simulink model "ps_model"  (R2025b)
settings: Solver=ode23tb  StartTime=0.0  StopTime=simlength  FixedStep=tc  MaxStep=tc
values from neighbouring files (symbols this model uses):
  omega_grid_emulator_nom = w_grid    (= 314.159265359)    [grid_emulator.m]
  omega_grid_nom = w_grid    (= 314.159265359)    [grid_emulator.m]
  ugrid_factor = 1    [grid_emulator.m]
  V_phase_normalization_factor = Vgrid_phase_normalization_factor    [grid_emulator.m]
  Vdc_base = 720    [grid_emulator.m]
  vn_eta_pu = 0    [grid_emulator.m]
  vn_xi_pu = 0    [grid_emulator.m]
  vp_xi_pu = 1    [grid_emulator.m]
undefined symbols (not defined in the file or in its folder): CFi, fnom, fPWM_INV, i_nom, ki_i, ki_u, kp_i, kp_u, Ld2_trafo_out, magnitude, n10, number_of_cells, omega_nom, Q, q1Kalman, q2Kalman, q3Kalman, R_RLload, Rd2_trafo_out, rKalman, tc, time_load_step, ts_afe, ts_inv, tsample, u_nom, Vdc_nom
libraries: fl_lib x120, nesl_utility x67, ee_lib x7, cstblocks x4, moving_average_filter x4, single_phase_transformer_lib x3, lithium_ion_cell_lib x1, simulink x1, threephase_inductor_lib x1
(part 4 of 4)

== system ps_model/inverter/MOS based inverter/spwm/modulator1/PWM generator 3 ==
  m_index : Inport
  phase : Inport  Port=2
  Clock : Clock
  Constant : Constant  Value=dead_time*f
  Constant1 : Constant  Value=polarity
  Constant2 : Constant  Value=1/f
  Constant4 : Constant
  Data Type Conversion1 : DataTypeConversion
  Data Type Conversion2 : DataTypeConversion
  Gain4 : Gain  Gain=1/2
  Gain5 : Gain  Gain=1/(pi/2)
  Hit Crossing : HitCross  ShowOutputPort=off
  Hit Crossing1 : HitCross  ShowOutputPort=off
  MATLAB Function : MATLAB Function  TreatAsAtomicUnit=on
  Relational Operator1 : RelationalOperator  Operator=<=  InputSameDT=off
  Relational Operator2 : RelationalOperator  Operator=<=  InputSameDT=off
  Relay : Relay  OnOutputValue=pos_cmd_gate  OffOutputValue=neg_cmd_gate
  Relay1 : Relay  OnOutputValue=pos_cmd_gate  OffOutputValue=neg_cmd_gate
  Saturation1 : Saturate  UpperLimit=m_up  LowerLimit=m_low
  Sum : Sum  Inputs=|++  SaturateOnIntegerOverflow=on
  Sum1 : Sum  Inputs=-+|  SaturateOnIntegerOverflow=on
  Sum3 : Sum  Inputs=|++
  Switch : Switch  Criteria=u2 > Threshold  SaturateOnIntegerOverflow=off  InputSameDT=off
  Switch1 : Switch  Criteria=u2 > Threshold  SaturateOnIntegerOverflow=off  InputSameDT=off
  m1 : Outport
  m2 : Outport  Port=2
  wires:
  Relay1/1 -> m1/1
  Switch1/1 -> Relay1/1
  Constant1/1 -> Switch/2, Switch1/2
  Relay/1 -> m2/1
  Constant4/1 -> Sum3/2
  Sum3/1 -> Gain4/1
  Gain5/1 -> Sum3/1
  MATLAB Function/1(y) -> Gain5/1
  phase/1 -> MATLAB Function/2(phase)
  Constant2/1 -> MATLAB Function/3(period)
  Clock/1 -> MATLAB Function/1(t)
  Switch/1 -> Relay/1
  Data Type Conversion1/1 -> Switch1/1, Switch/3, Hit Crossing/1
  Gain4/1 -> Relational Operator1/2, Relational Operator2/1
  Sum1/1 -> Relational Operator2/2
  Sum/1 -> Relational Operator1/1
  Saturation1/1 -> Sum1/2, Sum/1
  Constant/1 -> Sum1/1, Sum/2
  Data Type Conversion2/1 -> Hit Crossing1/1, Switch1/3, Switch/1
  Relational Operator2/1 -> Data Type Conversion2/1
  m_index/1 -> Saturation1/1
  Relational Operator1/1 -> Data Type Conversion1/1

== system ps_model/inverter/MOS based inverter/sv_pwm/modulator1/PWM generator 1 ==
  m_index : Inport
  phase : Inport  Port=2
  Clock : Clock
  Constant : Constant  Value=dead_time*f
  Constant1 : Constant  Value=polarity
  Constant2 : Constant  Value=1/f
  Constant4 : Constant
  Data Type Conversion1 : DataTypeConversion
  Data Type Conversion2 : DataTypeConversion
  Gain4 : Gain  Gain=1/2
  Gain5 : Gain  Gain=1/(pi/2)
  Hit Crossing : HitCross  ShowOutputPort=off
  Hit Crossing1 : HitCross  ShowOutputPort=off
  MATLAB Function : MATLAB Function  TreatAsAtomicUnit=on
  Relational Operator1 : RelationalOperator  Operator=<=  InputSameDT=off
  Relational Operator2 : RelationalOperator  Operator=<=  InputSameDT=off
  Relay : Relay  OnOutputValue=pos_cmd_gate  OffOutputValue=neg_cmd_gate
  Relay1 : Relay  OnOutputValue=pos_cmd_gate  OffOutputValue=neg_cmd_gate
  Saturation1 : Saturate  UpperLimit=m_up  LowerLimit=m_low
  Sum : Sum  Inputs=|++  SaturateOnIntegerOverflow=on
  Sum1 : Sum  Inputs=-+|  SaturateOnIntegerOverflow=on
  Sum3 : Sum  Inputs=|++
  Switch : Switch  Criteria=u2 > Threshold  SaturateOnIntegerOverflow=off  InputSameDT=off
  Switch1 : Switch  Criteria=u2 > Threshold  SaturateOnIntegerOverflow=off  InputSameDT=off
  m1 : Outport
  m2 : Outport  Port=2
  wires:
  Relational Operator1/1 -> Data Type Conversion1/1
  m_index/1 -> Saturation1/1
  Relational Operator2/1 -> Data Type Conversion2/1
  Data Type Conversion2/1 -> Switch/1, Switch1/3, Hit Crossing1/1
  Constant/1 -> Sum/2, Sum1/1
  Saturation1/1 -> Sum/1, Sum1/2
  Sum/1 -> Relational Operator1/1
  Sum1/1 -> Relational Operator2/2
  Gain4/1 -> Relational Operator2/1, Relational Operator1/2
  Data Type Conversion1/1 -> Hit Crossing/1, Switch/3, Switch1/1
  Switch/1 -> Relay/1
  Clock/1 -> MATLAB Function/1(t)
  Constant2/1 -> MATLAB Function/3(period)
  phase/1 -> MATLAB Function/2(phase)
  MATLAB Function/1(y) -> Gain5/1
  Gain5/1 -> Sum3/1
  Sum3/1 -> Gain4/1
  Constant4/1 -> Sum3/2
  Relay/1 -> m2/1
  Constant1/1 -> Switch1/2, Switch/2
  Switch1/1 -> Relay1/1
  Relay1/1 -> m1/1

== system ps_model/inverter/MOS based inverter/sv_pwm/modulator1/PWM generator 2 ==
  m_index : Inport
  phase : Inport  Port=2
  Clock : Clock
  Constant : Constant  Value=dead_time*f
  Constant1 : Constant  Value=polarity
  Constant2 : Constant  Value=1/f
  Constant4 : Constant
  Data Type Conversion1 : DataTypeConversion
  Data Type Conversion2 : DataTypeConversion
  Gain4 : Gain  Gain=1/2
  Gain5 : Gain  Gain=1/(pi/2)
  Hit Crossing : HitCross  ShowOutputPort=off
  Hit Crossing1 : HitCross  ShowOutputPort=off
  MATLAB Function : MATLAB Function  TreatAsAtomicUnit=on
  Relational Operator1 : RelationalOperator  Operator=<=  InputSameDT=off
  Relational Operator2 : RelationalOperator  Operator=<=  InputSameDT=off
  Relay : Relay  OnOutputValue=pos_cmd_gate  OffOutputValue=neg_cmd_gate
  Relay1 : Relay  OnOutputValue=pos_cmd_gate  OffOutputValue=neg_cmd_gate
  Saturation1 : Saturate  UpperLimit=m_up  LowerLimit=m_low
  Sum : Sum  Inputs=|++  SaturateOnIntegerOverflow=on
  Sum1 : Sum  Inputs=-+|  SaturateOnIntegerOverflow=on
  Sum3 : Sum  Inputs=|++
  Switch : Switch  Criteria=u2 > Threshold  SaturateOnIntegerOverflow=off  InputSameDT=off
  Switch1 : Switch  Criteria=u2 > Threshold  SaturateOnIntegerOverflow=off  InputSameDT=off
  m1 : Outport
  m2 : Outport  Port=2
  wires:
  Relay1/1 -> m1/1
  Switch1/1 -> Relay1/1
  Constant1/1 -> Switch/2, Switch1/2
  Relay/1 -> m2/1
  Constant4/1 -> Sum3/2
  Sum3/1 -> Gain4/1
  Gain5/1 -> Sum3/1
  MATLAB Function/1(y) -> Gain5/1
  phase/1 -> MATLAB Function/2(phase)
  Constant2/1 -> MATLAB Function/3(period)
  Clock/1 -> MATLAB Function/1(t)
  Switch/1 -> Relay/1
  Data Type Conversion1/1 -> Switch1/1, Switch/3, Hit Crossing/1
  Gain4/1 -> Relational Operator1/2, Relational Operator2/1
  Sum1/1 -> Relational Operator2/2
  Sum/1 -> Relational Operator1/1
  Saturation1/1 -> Sum1/2, Sum/1
  Constant/1 -> Sum1/1, Sum/2
  Data Type Conversion2/1 -> Hit Crossing1/1, Switch1/3, Switch/1
  Relational Operator2/1 -> Data Type Conversion2/1
  m_index/1 -> Saturation1/1
  Relational Operator1/1 -> Data Type Conversion1/1

== system ps_model/inverter/MOS based inverter/sv_pwm/modulator1/PWM generator 3 ==
  m_index : Inport
  phase : Inport  Port=2
  Clock : Clock
  Constant : Constant  Value=dead_time*f
  Constant1 : Constant  Value=polarity
  Constant2 : Constant  Value=1/f
  Constant4 : Constant
  Data Type Conversion1 : DataTypeConversion
  Data Type Conversion2 : DataTypeConversion
  Gain4 : Gain  Gain=1/2
  Gain5 : Gain  Gain=1/(pi/2)
  Hit Crossing : HitCross  ShowOutputPort=off
  Hit Crossing1 : HitCross  ShowOutputPort=off
  MATLAB Function : MATLAB Function  TreatAsAtomicUnit=on
  Relational Operator1 : RelationalOperator  Operator=<=  InputSameDT=off
  Relational Operator2 : RelationalOperator  Operator=<=  InputSameDT=off
  Relay : Relay  OnOutputValue=pos_cmd_gate  OffOutputValue=neg_cmd_gate
  Relay1 : Relay  OnOutputValue=pos_cmd_gate  OffOutputValue=neg_cmd_gate
  Saturation1 : Saturate  UpperLimit=m_up  LowerLimit=m_low
  Sum : Sum  Inputs=|++  SaturateOnIntegerOverflow=on
  Sum1 : Sum  Inputs=-+|  SaturateOnIntegerOverflow=on
  Sum3 : Sum  Inputs=|++
  Switch : Switch  Criteria=u2 > Threshold  SaturateOnIntegerOverflow=off  InputSameDT=off
  Switch1 : Switch  Criteria=u2 > Threshold  SaturateOnIntegerOverflow=off  InputSameDT=off
  m1 : Outport
  m2 : Outport  Port=2
  wires:
  Relational Operator1/1 -> Data Type Conversion1/1
  m_index/1 -> Saturation1/1
  Relational Operator2/1 -> Data Type Conversion2/1
  Data Type Conversion2/1 -> Switch/1, Switch1/3, Hit Crossing1/1
  Constant/1 -> Sum/2, Sum1/1
  Saturation1/1 -> Sum/1, Sum1/2
  Sum/1 -> Relational Operator1/1
  Sum1/1 -> Relational Operator2/2
  Gain4/1 -> Relational Operator2/1, Relational Operator1/2
  Data Type Conversion1/1 -> Hit Crossing/1, Switch/3, Switch1/1
  Switch/1 -> Relay/1
  Clock/1 -> MATLAB Function/1(t)
  Constant2/1 -> MATLAB Function/3(period)
  phase/1 -> MATLAB Function/2(phase)
  MATLAB Function/1(y) -> Gain5/1
  Gain5/1 -> Sum3/1
  Sum3/1 -> Gain4/1
  Constant4/1 -> Sum3/2
  Relay/1 -> m2/1
  Constant1/1 -> Switch1/2, Switch/2
  Switch1/1 -> Relay1/1
  Relay1/1 -> m1/1

== matlab function ps_model/inverter/MOS based inverter/spwm/modulator1/PWM generator 3/MATLAB Function ==
  data: t input; y output; phase input; period input
function y = trgo(t,phase,period)
x = sin(2*pi/period*t - phase -pi/2);
y = asin(x);

== matlab function ps_model/battery_system/battery_system/LithiumIonBattery/SOC_estimator/Kalman_observer/lithium-ion battery model ==
  data: i input; SOC output; u output; ts input; Q input; l1 input; l2 input; l3 input; vout input; x output
function [SOC, u, x] = lithium_ion_battery(i,ts,Q,l1,l2,l3,vout)

    persistent z_po ir_po h_po vout_hat

    if isempty(z_po)
        ir_po = 0;
        h_po = 0;
        z_po = 0.35;        
    end
    
        R0 = 0.15;
        R = 0.15;
        C = 0.1;
        M = 125;
        E_1 = -1.031;
        E0 = 3.685;
        E1 = 0.2156;
        E2 = 0;
        E3 = 0;
        Elog = -0.05;
        alpha = 35;
        N = 100;
        
        z_pr = z_po - ts/Q*i ;
    
        ir_pr = exp(-ts/(R*C))*ir_po + (1-exp(-ts/(R*C)))*i;

        h_pr = exp(-abs(i)*ts/Q)*h_po - (1-exp(-abs(i)*ts/Q))*sign(i);
        
        OCV = E_1*exp(-z_pr*alpha) + E0 + E1*z_pr + E2*z_pr^2 + E3*z_pr^3 + Elog*log(1-z_pr+ts);
        
        vout_hat = OCV*N + M*h_pr - R*ir_pr - R0*i;
        
        z_po = z_pr + l1*(vout - vout_hat);
        ir_po = ir_pr + l2*(vout - vout_hat);
        h_po = h_pr + l3*(vout - vout_hat);
        u = vout_hat;
        
        x = [z_po; ir_po; h_po];

    SOC = z_po;
end

== matlab function ps_model/control_system/current_measure/current_transformation/alphabeta2dq ==
  data: alpha input; d output; beta input; phase input; q output
function [d,q] = alphabeta2dq(alpha,beta,phase)

    d  =  alpha*cos(phase) + beta*sin(phase);
    q = -alpha*sin(phase) + beta*cos(phase);

end

== matlab function ps_model/inverter/MOS based inverter/spwm/uvw2alphabeta ==
  data: alpha input; u output; beta input; v output; w output
function [u,v,w] = alphabeta2uvw(alpha,beta)

u  = alpha;
v  = -0.5*alpha+sqrt(3)/2*beta;
w  = -0.5*alpha-sqrt(3)/2*beta;

end

== matlab function ps_model/inverter/MOS based inverter/sv_pwm/modulator1/PWM generator 1/MATLAB Function ==
  data: t input; y output; phase input; period input
function y = trgo(t,phase,period)
x = sin(2*pi/period*t - phase -pi/2);
y = asin(x);

== matlab function ps_model/control_system/current_measure/current_transformation/uvw2alphabeta ==
  data: u input; alpha output; v input; w input; beta output
function [alpha,beta] = uvw2alphabeta(u,v,w)

alpha = 2/3*(u - 1/2*v - 1/2*w);
beta  = 2/3*(sqrt(3)/2*(v - w));

end

== matlab function ps_model/control_system/dq2alphabeta ==
  data: d input; alpha output; q input; phase input; beta output
function [alpha,beta] = dq2alphabeta(d,q,phase)

    alpha  =  d*cos(phase) - q*sin(phase);
    beta = d*sin(phase) + q*cos(phase);

end

== matlab function ps_model/inverter/MOS based inverter/spwm/conditioning ==
  data: u1 input; u2 output; v1 input; v2 output; w2 output; w1 input
function [u2,v2,w2] = scaling(u1,v1,w1)

u2  = (u1+1)/2;
v2  = (v1+1)/2;
w2  = (w1+1)/2;

end

== matlab function ps_model/control_system/phase_gen/bounder1 ==
  data: u input; y output
function y = bounder(u)
    
    y = -pi + mod(u+3*pi,2*pi);
end

== matlab function ps_model/inverter/MOS based inverter/sv_pwm/modulator1/PWM generator 2/MATLAB Function ==
  data: t input; y output; phase input; period input
function y = trgo(t,phase,period)
x = sin(2*pi/period*t - phase -pi/2);
y = asin(x);

== matlab function ps_model/grid/grid_emulator/grid_emulator/phase_gen/bounder1 ==
  data: u input; y output
function y = bounder(u)    
    y = -pi + mod(u+3*pi,2*pi);
end

== matlab function ps_model/grid/grid_emulator/grid_emulator/voltage_reference/alphabeta2abc ==
  data: alpha input; a output; beta input; b output; c output
function [a,b,c] = alphabeta2abc(alpha,beta)

    a  =  alpha;
    b  =  -0.5*alpha + sqrt(3)/2*beta;
    c  =  -0.5*alpha - sqrt(3)/2*beta;
end

== matlab function ps_model/grid/grid_emulator/grid_emulator/voltage_reference/xieta2alphabeta_neg ==
  data: xi input; alpha output; eta input; gamma input; beta output
function [alpha,beta] = xieta2alphabeta_neg(xi,eta,gamma)

    alpha  =  xi*cos(gamma) + eta*sin(gamma);
    beta = -xi*sin(gamma) + eta*cos(gamma);

end

== matlab function ps_model/grid/grid_emulator/grid_emulator/voltage_reference/xieta2alphabeta_pos ==
  data: xi input; alpha output; eta input; gamma input; beta output
function [alpha,beta] = xieta2alphabeta_pos(xi,eta,gamma)

    alpha  =  xi*cos(gamma) - eta*sin(gamma);
    beta = xi*sin(gamma) + eta*cos(gamma);

end

== matlab function ps_model/inverter/MOS based inverter/sv_pwm/modulator1/PWM generator 3/MATLAB Function ==
  data: t input; y output; phase input; period input
function y = trgo(t,phase,period)
x = sin(2*pi/period*t - phase -pi/2);
y = asin(x);

== matlab function ps_model/control_system/voltage_measure/voltage_transformation/alphabeta2dq ==
  data: alpha input; d output; beta input; phase input; q output
function [d,q] = alphabeta2dq(alpha,beta,phase)

    d  =  alpha*cos(phase) + beta*sin(phase);
    q = -alpha*sin(phase) + beta*cos(phase);

end

== matlab function ps_model/battery_system/battery_system/LithiumIonBattery/SOC_estimator/Kalman_observer/kalman_observer_gains ==
  data: i input; ts input; l1 output; z input; q1 input; q2 input; q3 input; r input; Q input; l2 output; l3 output
function [l1,l2,l3] = EKF(i,ts,z,q1,q2,q3,r,Q)

    persistent  p11 p12 p13 p21 p22 p23 p31 p32 p33

    if isempty(p11)
        p11 = q1;
        p12 = 0;
        p13 = 0;
        p21 = 0;
        p22 = q2;
        p23 = 0;
        p31 = 0;
        p32 = 0;
        p33 = q3;
    end
    R = 0.15;
    C = 10;
    M = 125;
    E_1 = -1.031;
    E1 = 0.2156;
    E2 = 0;
    E3 = 0;
    Elog = -0.05;
    alpha = 35;

    a11 = 1;
    a12 = 0;
    a13 = 0;
    a21 = 0;
    a22 = exp(-ts/(R*C));
    a23 = 0;
    a31 = 0;
    a32 = 0;
    a33 = abs(exp(-i*ts/Q));

    c1 = -alpha*E_1*abs(exp(-alpha*z)) + E1 + 2*E2*z + 3*E3*z^2 - Elog/(1-z+ts);
    c2 = -R;
    c3 = M;
    
    p11_pr = a11*(a11*p11 + a12*p21 + a13*p31) + a12*(a11*p12 + a12*p22 + a13*p32) + a13*(a11*p13 + a12*p23 + a13*p33) + q1;

    p12_pr = a21*(a11*p11 + a12*p21 + a13*p31) + a22*(a11*p12 + a12*p22 + a13*p32) + a23*(a11*p13 + a12*p23 + a13*p33);

    p13_pr = a31*(a11*p11 + a12*p21 + a13*p31) + a32*(a11*p12 + a12*p22 + a13*p32) + a33*(a11*p13 + a12*p23 + a13*p33);

    p21_pr = a11*(a21*p11 + a22*p21 + a23*p31) + a12*(a21*p12 + a22*p22 + a23*p32) + a13*(a21*p13 + a22*p23 + a23*p33);

    p22_pr = a21*(a21*p11 + a22*p21 + a23*p31) + a22*(a21*p12 + a22*p22 + a23*p32) + a23*(a21*p13 + a22*p23 + a23*p33) + q2;

    p23_pr = a31*(a21*p11 + a22*p21 + a23*p31) + a32*(a21*p12 + a22*p22 + a23*p32) + a33*(a21*p13 + a22*p23 + a23*p33);

    p31_pr = a11*(a31*p11 + a32*p21 + a33*p31) + a12*(a31*p12 + a32*p22 + a33*p32) + a13*(a31*p13 + a32*p23 + a33*p33);

    p32_pr = a21*(a31*p11 + a32*p21 + a33*p31) + a22*(a31*p12 + a32*p22 + a33*p32) + a23*(a31*p13 + a32*p23 + a33*p33);

    p33_pr = a31*(a31*p11 + a32*p21 + a33*p31) + a32*(a31*p12 + a32*p22 + a33*p32) + a33*(a31*p13 + a32*p23 + a33*p33) + q3;

    den = c1*(c1*p11 + c2*p21 + c3*p31) + c2*(c1*p12 + c2*p22 + c3*p32) + c3*(c1*p13 + c2*p23 + c3*p33) + r;
 
    l1 = (c1*p11 + c2*p12 + c3*p13)/den;
    l2 = (c1*p21 + c2*p22 + c3*p23)/den;
    l3 = (c1*p31 + c2*p32 + c3*p33)/den;
    
    p11 = (1 - c1*l1)*p11_pr - c2*l1*p21_pr - c3*l1*p31_pr;
    
    p12 = (1 - c1*l1)*p12_pr - c2*l1*p22_pr - c3*l1*p32_pr;
    
    p13 = (1 - c1*l1)*p13_pr - c2*l1*p23_pr - c3*l1*p33_pr;
    
    p21 = -c1*l2*p11_pr + (1 - c2*l2)*p21_pr - c3*l2*p31_pr;
    
    p22 = -c1*l2*p12_pr + (1 - c2*l2)*p22_pr - c3*l2*p32_pr;
    
    p23 = -c1*l2*p13_pr + (1 - c2*l2)*p23_pr - c3*l2*p33_pr;
    
    p31 = -c1*l3*p11_pr - c2*l3*p21_pr + (1 - c3*l3)*p31_pr;
    
    p32 = -c1*l3*p12_pr - c2*l3*p22_pr + (1 - c3*l3)*p32_pr;
    
    p33 = -c1*l3*p13_pr - c2*l3*p23_pr + (1 - c3*l3)*p33_pr;
end

== matlab function ps_model/control_system/voltage_measure/voltage_transformation/uvw2alphabeta ==
  data: u input; alpha output; v input; w input; beta output
function [alpha,beta] = uvw2alphabeta(u,v,w)

alpha = 2/3*(u - 1/2*v - 1/2*w);
beta  = 2/3*(sqrt(3)/2*(v - w));

end

== matlab function ps_model/inverter/MOS based inverter/spwm/modulator1/PWM generator 1/MATLAB Function ==
  data: t input; y output; phase input; period input
function y = trgo(t,phase,period)
x = sin(2*pi/period*t - phase -pi/2);
y = asin(x);

== matlab function ps_model/inverter/MOS based inverter/spwm/modulator1/PWM generator 2/MATLAB Function ==
  data: t input; y output; phase input; period input
function y = trgo(t,phase,period)
x = sin(2*pi/period*t - phase -pi/2);
y = asin(x);
